simulink model "W06_1_point"  (R2024b)
settings: Solver=ode4  StartTime=0  StopTime=120  FixedStep=h  RelTol=1e-3
InitFcn:
  | addpath(fullfile(fileparts(fileparts(fileparts(get_param(bdroot, 'FileName')))), '_tools'), fileparts(get_param(bdroot, 'FileName'))); run_alone('W06', bdroot);
StopFcn:
  | W06_plot;
values from neighbouring files (symbols this model uses):
  animate = 1    [W06_0_setup.m]    (also in W06_1_point_run.m = 0; W06_2_sway_run.m = 0; W06_3_thrust_run.m = 0; W06_4_stop_run.m = 0)
  beta_c = pi/2    (= 1.57079632679)    [W06_0_setup.m]    (also in W06_4_stop_run.m = V.beta_c)
  Binv = inv(B)    [W06_0_setup.m]
  bow = [l_f, k_bow, n_bow_max]    [W06_0_setup.m]
  h = 0.02    [W06_0_setup.m]
  k_bow = cfg.k_bow    [W06_0_setup.m]
  k_neg = cfg.k_neg    [W06_0_setup.m]
  k_pos = cfg.k_pos    [W06_0_setup.m]
  Kb = 1    [W06_0_setup.m]
  Kd = 100    [W06_0_setup.m]
  Ki_u = 200    [W06_0_setup.m]
  Ki_v = 120    [W06_0_setup.m]
  Kp = 300    [W06_0_setup.m]
  Kp_pos = 0.30    (= 0.3)    [W06_0_setup.m]    (also in W06_4_stop_run.m = V.Kp_pos)
  Kp_u = 200    [W06_0_setup.m]
  Kp_v = 150    [W06_0_setup.m]
  mp = 25    [W06_0_setup.m]
  n_bow_max = cfg.n_bow_max    [W06_0_setup.m]    (also in W06_1_point_run.m = V.n_bow_max)
  n_max = cfg.n_max    [W06_0_setup.m]
  N_max = 2*y_pont*min(T_max, -T_min)    [W06_0_setup.m]
  n_min = cfg.n_min    [W06_0_setup.m]
  psi_d_cmd = 0    [W06_0_setup.m]    (also in W06_1_point_run.m; W06_8_ned_run.m)
  rp = [0.05 0 -0.35]'    [W06_0_setup.m]
  u_lim = 0.80    (= 0.8)    [W06_0_setup.m]
  V_c = 0    [W06_0_setup.m]    (also in W06_4_stop_run.m = V.V_c)
  v_lim = 0.35    [W06_0_setup.m]
  x0 = zeros(12,1)    [W06_0_setup.m]
  X_max = 120    [W06_0_setup.m]    (also in W06_plot.m = base_var('X_max', 120))
  Y_max = min(abs(T_min)/(l_f/(2*y_pont)), F_B_max)    [W06_0_setup.m]    (also in W06_plot.m = base_var('Y_max', 35.13))
settings Model: Creator=admin  LastModifiedBy=admin
settings DataIOCC: ReturnWorkspaceOutputs=off

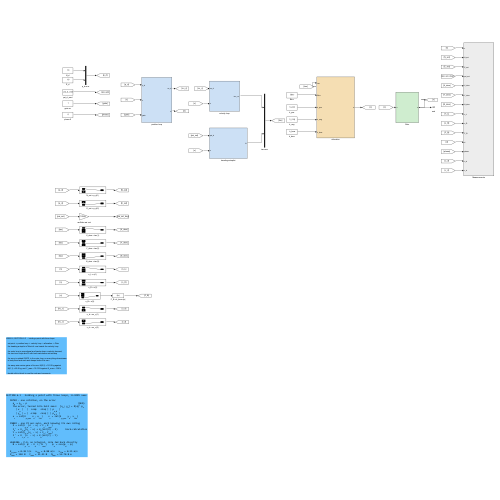
[thumbnail: Simulink's stored preview of the top-level diagram]
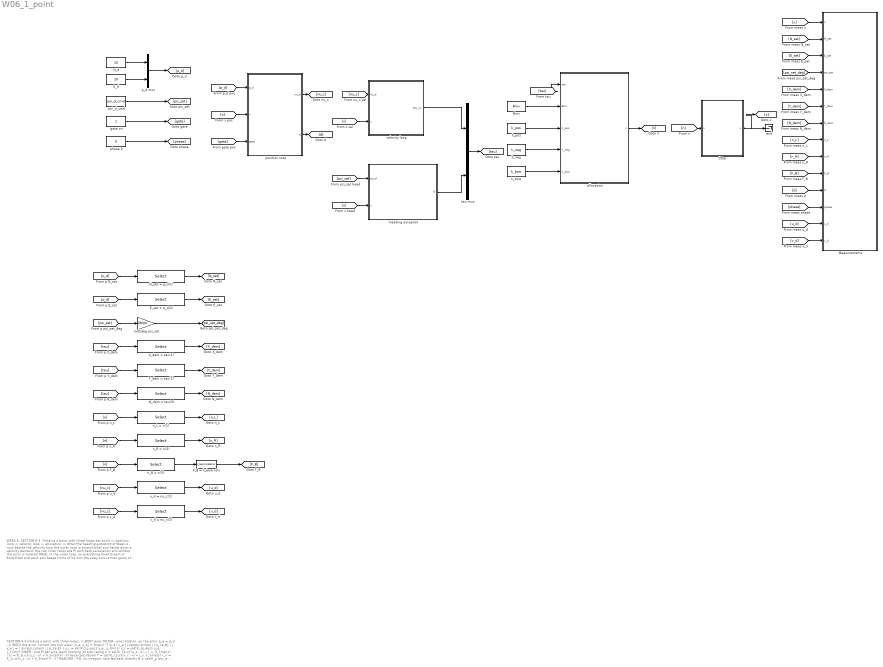
== system W06_1_point ==
  note: WEEK 6, SECTION 6-3  -  holding a point with three loops
      |
      |    set point -> position loop -> velocity loop -> allocation -> Otter
      |    the heading autopilot of Week 4 runs beside the velocity loop
      |
      |    the outer loop is proportional and hands down a velocity demand;
      |    the two inner loops are PI with back-calculation anti-windup
      |
      |    the error is rotated ONCE, in the outer loop, so everything downstream
      |    is body-fixed and each axis keeps limits of its own
      |
      |    the sway axis carries gains of its own: M(2,2) = 162.5 kg against
      |    M(1,1) = 85.5 kg, and Y_max = 35.13 N against X_max = 120 N
      |
      |    double-click a block to read its code and comments
  note: SECTION 6-3   holding a point with three loops, in BODY axes
      |
      |    OUTER - one rotation, on the error
      |      p_e = p_d - p                                      (NED)
      |      the error, turned into hull axes:  [x_e; y_e] = R(\psi)^T p_e
      |        | x_e |   |  cos\psi   sin\psi | | p_{e,N} |
      |        | y_e | = | -sin\psi   cos\psi | | p_{e,E} |
      |      u_c = sat(K_{p,pos} x_e, u_{lim})    v_c = sat(K_{p,pos} y_e, v_{lim})
      |
      |    INNER - one PI per axis, each knowing its own rating
      |      X = sat(K_{p,u}(u_c - u) + I_u, X_{max})
      |      I_u' = K_{i,u}(u_c - u) + K_b(sat(X) - X)      back-calculation
      |      Y = sat(K_{p,v}(v_c - v) + I_v, Y_{max})
      |      I_v' = K_{i,v}(v_c - v) + K_b(sat(Y) - Y)
      |
      |    HEADING - P-D, no integral, rate fed back directly
      |      N = sat(K_p \psi_e - K_d r, N_{max})    \psi_e = ssa(\psi_d - \psi)
      |
      |    K_{p,pos} = 0.30 1/s   u_{lim} = 0.80 m/s   v_{lim} = 0.35 m/s
      |    X_{max} = 120 N   Y_{max} = 35.13 N   N_{max} = 52.70 N m
  Binv : Constant  Value=Binv
  E_d : Constant  Value=10
  E_set = p_d(2) : Selector  InputPortWidth=2  IndexOptions=Index vector (dialog)  Indices=2  OutputSizes=1
  F_B = k_bow n|n| : Fcn  Expr=k_bow*u*abs(u)
  Measurements : Subsystem
  N_d : Constant  Value=10
  N_dem = tau(3) : Selector  InputPortWidth=3  IndexOptions=Index vector (dialog)  Indices=3  OutputSizes=1
  N_set = p_d(1) : Selector  InputPortWidth=2  IndexOptions=Index vector (dialog)  Indices=1  OutputSizes=1
  Otter : Subsystem
  X_dem = tau(1) : Selector  InputPortWidth=3  IndexOptions=Index vector (dialog)  Indices=1  OutputSizes=1
  Y_dem = tau(2) : Selector  InputPortWidth=3  IndexOptions=Index vector (dialog)  Indices=2  OutputSizes=1
  allocation : Subsystem
  end : Terminator
  gate on : Constant
  heading autopilot : Subsystem
  k_bow : Constant  Value=k_bow
  k_neg : Constant  Value=k_neg
  k_pos : Constant  Value=k_pos
  n_B = n(3) : Selector  InputPortWidth=3  IndexOptions=Index vector (dialog)  Indices=3  OutputSizes=1
  n_L = n(1) : Selector  InputPortWidth=3  IndexOptions=Index vector (dialog)  Indices=1  OutputSizes=1
  n_R = n(2) : Selector  InputPortWidth=3  IndexOptions=Index vector (dialog)  Indices=2  OutputSizes=1
  p_d mux : Mux  Inputs=2
  phase 0 : Constant  Value=0
  position loop : Subsystem
  psi_d_cmd : Constant  Value=psi_d_cmd
  rad2deg psi_set : Gain  Gain=180/pi
  tau mux : Mux  Inputs=2
  u_d = nu_c(1) : Selector  InputPortWidth=2  IndexOptions=Index vector (dialog)  Indices=1  OutputSizes=1
  v_d = nu_c(2) : Selector  InputPortWidth=2  IndexOptions=Index vector (dialog)  Indices=2  OutputSizes=1
  velocity loop : Subsystem
  wires:
  N_d/1 -> p_d mux/1
  E_d/1 -> p_d mux/2
  p_d mux/1 -> [p_d]
  psi_d_cmd/1 -> [psi_set]
  gate on/1 -> [gate]
  phase 0/1 -> [phase]
  [p_d] -> position loop/1(p_d)
  [x] -> position loop/2(x)
  [gate] -> position loop/3(gate)
  position loop/2(d) -> [d]
  position loop/1(nu_d) -> [nu_c]
  [nu_c] -> velocity loop/1(nu_d)
  [x] -> velocity loop/2(x)
  [psi_set] -> heading autopilot/1(psi_d)
  [x] -> heading autopilot/2(x)
  velocity loop/1(tau_uv) -> tau mux/1
  heading autopilot/1(N) -> tau mux/2
  tau mux/1 -> [tau]
  [tau] -> allocation/1(tau)
  Binv/1 -> allocation/2(Binv)
  k_pos/1 -> allocation/3(k_pos)
  k_neg/1 -> allocation/4(k_neg)
  k_bow/1 -> allocation/5(k_bow)
  allocation/1(n) -> [n]
  [n] -> Otter/1(n)
  Otter/1(x) -> [x], end/1
  [x] -> Measurements/1(x)
  [N_set] -> Measurements/2(N_set)
  [E_set] -> Measurements/3(E_set)
  [psi_set_deg] -> Measurements/4(psi_set)
  [X_dem] -> Measurements/5(X_dem)
  [Y_dem] -> Measurements/6(Y_dem)
  [N_dem] -> Measurements/7(N_dem)
  [n_L] -> Measurements/8(n_L)
  [n_R] -> Measurements/9(n_R)
  [F_B] -> Measurements/10(F_B)
  [d] -> Measurements/11(d)
  [phase] -> Measurements/12(phase)
  [u_d] -> Measurements/13(u_d)
  [v_d] -> Measurements/14(v_d)
  [p_d] -> N_set = p_d(1)/1
  N_set = p_d(1)/1 -> [N_set]
  [p_d] -> E_set = p_d(2)/1
  E_set = p_d(2)/1 -> [E_set]
  [psi_set] -> rad2deg psi_set/1
  rad2deg psi_set/1 -> [psi_set_deg]
  [tau] -> X_dem = tau(1)/1
  X_dem = tau(1)/1 -> [X_dem]
  [tau] -> Y_dem = tau(2)/1
  Y_dem = tau(2)/1 -> [Y_dem]
  [tau] -> N_dem = tau(3)/1
  N_dem = tau(3)/1 -> [N_dem]
  [n] -> n_L = n(1)/1
  n_L = n(1)/1 -> [n_L]
  [n] -> n_R = n(2)/1
  n_R = n(2)/1 -> [n_R]
  [n] -> n_B = n(3)/1
  n_B = n(3)/1 -> F_B = k_bow n|n|/1
  F_B = k_bow n|n|/1 -> [F_B]
  [nu_c] -> u_d = nu_c(1)/1
  u_d = nu_c(1)/1 -> [u_d]
  [nu_c] -> v_d = nu_c(2)/1
  v_d = nu_c(2)/1 -> [v_d]

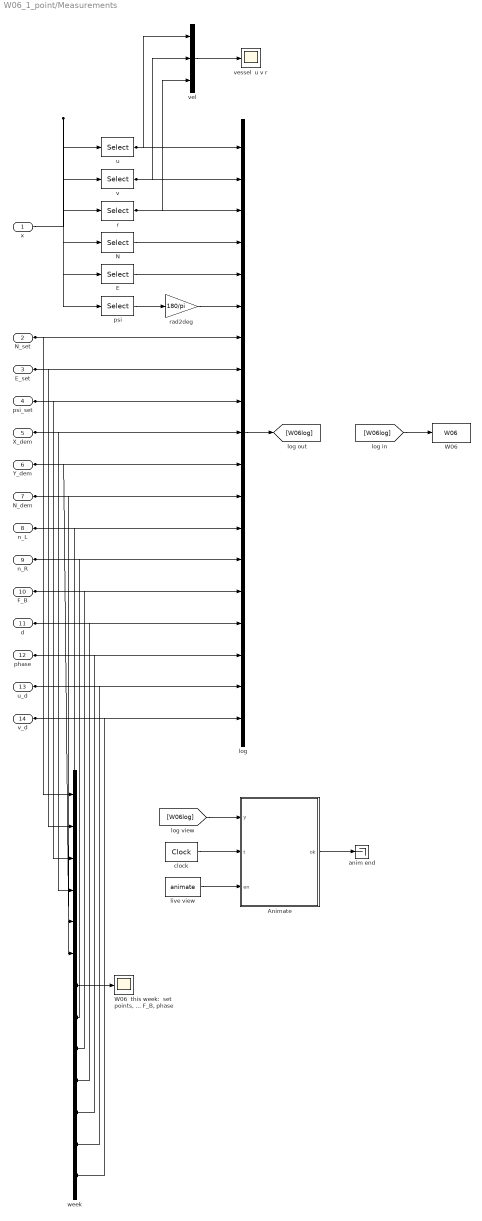
== system W06_1_point/Measurements ==
  x : Inport
  N_set : Inport  Port=2
  E_set : Inport  Port=3
  psi_set : Inport  Port=4
  X_dem : Inport  Port=5
  Y_dem : Inport  Port=6
  N_dem : Inport  Port=7
  n_L : Inport  Port=8
  n_R : Inport  Port=9
  F_B : Inport  Port=10
  d : Inport  Port=11
  phase : Inport  Port=12
  u_d : Inport  Port=13
  v_d : Inport  Port=14
  Animate : MATLAB Function  TreatAsAtomicUnit=on
  E : Selector  InputPortWidth=12  IndexOptions=Index vector (dialog)  Indices=8  OutputSizes=1
  N : Selector  InputPortWidth=12  IndexOptions=Index vector (dialog)  Indices=7  OutputSizes=1
  W06 : ToWorkspace  VariableName=W06  SaveFormat=Structure With Time  SampleTime=-1
  "W06  this week:  set points, demands, n_L n_R, F_B, phase" : Scope
  anim end : Terminator
  clock : DigitalClock  SampleTime=h
  live view : Constant  Value=animate
  log : Mux  Inputs=19
  psi : Selector  InputPortWidth=12  IndexOptions=Index vector (dialog)  Indices=12  OutputSizes=1
  r : Selector  InputPortWidth=12  IndexOptions=Index vector (dialog)  Indices=6  OutputSizes=1
  rad2deg : Gain  Gain=180/pi
  u : Selector  InputPortWidth=12  IndexOptions=Index vector (dialog)  Indices=1  OutputSizes=1
  v : Selector  InputPortWidth=12  IndexOptions=Index vector (dialog)  Indices=2  OutputSizes=1
  vel : Mux  Inputs=3
  vessel  u v r : Scope
  week : Mux  Inputs=13
  wires:
  x/1 -> u/1, v/1, r/1, N/1, E/1, psi/1
  log/1 -> [W06log]
  [W06log] -> W06/1
  psi/1 -> rad2deg/1
  u/1 -> log/1, vel/1
  v/1 -> log/2, vel/2
  r/1 -> log/3, vel/3
  N/1 -> log/4
  E/1 -> log/5
  rad2deg/1 -> log/6
  N_set/1 -> log/7, week/1
  E_set/1 -> log/8, week/2
  psi_set/1 -> log/9, week/3
  X_dem/1 -> log/10, week/4
  Y_dem/1 -> log/11, week/5
  N_dem/1 -> log/12, week/6
  n_L/1 -> log/13, week/7
  n_R/1 -> log/14, week/8
  F_B/1 -> log/15, week/9
  d/1 -> log/16, week/10
  phase/1 -> log/17, week/11
  u_d/1 -> log/18, week/12
  v_d/1 -> log/19, week/13
  vel/1 -> vessel  u v r/1
  week/1 -> "W06  this week:  set points, demands, n_L n_R, F_B, phase"/1
  [W06log] -> Animate/1(y)
  clock/1 -> Animate/2(t)
  live view/1 -> Animate/3(en)
  Animate/1(ok) -> anim end/1

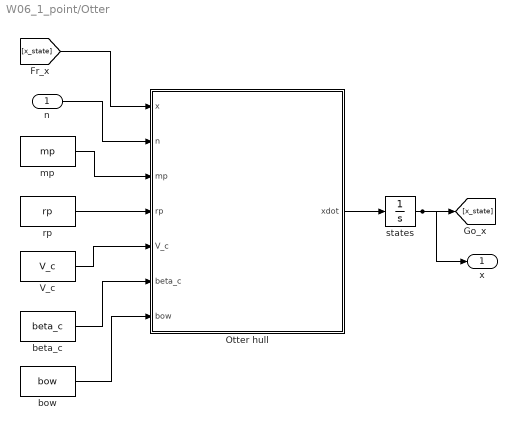
== system W06_1_point/Otter ==
  n : Inport
  Otter hull : MATLAB Function  TreatAsAtomicUnit=on
  V_c : Constant  Value=V_c
  beta_c : Constant  Value=beta_c
  bow : Constant  Value=bow
  mp : Constant  Value=mp
  rp : Constant  Value=rp
  states : Integrator  InitialCondition=x0
  x : Outport
  wires:
  [x_state] -> Otter hull/1(x)
  bow/1 -> Otter hull/7(bow)
  rp/1 -> Otter hull/4(rp)
  n/1 -> Otter hull/2(n)
  Otter hull/1(xdot) -> states/1
  mp/1 -> Otter hull/3(mp)
  V_c/1 -> Otter hull/5(V_c)
  beta_c/1 -> Otter hull/6(beta_c)
  states/1 -> [x_state], x/1

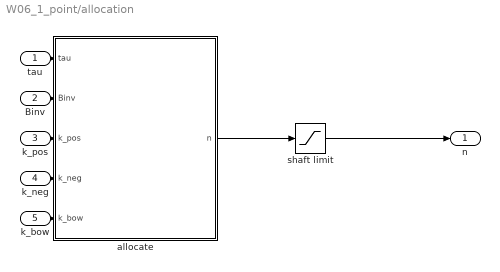
== system W06_1_point/allocation ==
  tau : Inport
  Binv : Inport  Port=2
  k_pos : Inport  Port=3
  k_neg : Inport  Port=4
  k_bow : Inport  Port=5
  allocate : MATLAB Function  TreatAsAtomicUnit=on
  shaft limit : Saturate  UpperLimit="[ n_max;  n_max;  n_bow_max]"  LowerLimit="[ n_min;  n_min; -n_bow_max]"
  n : Outport
  wires:
  tau/1 -> allocate/1(tau)
  Binv/1 -> allocate/2(Binv)
  k_pos/1 -> allocate/3(k_pos)
  k_neg/1 -> allocate/4(k_neg)
  k_bow/1 -> allocate/5(k_bow)
  allocate/1(n) -> shaft limit/1
  shaft limit/1 -> n/1

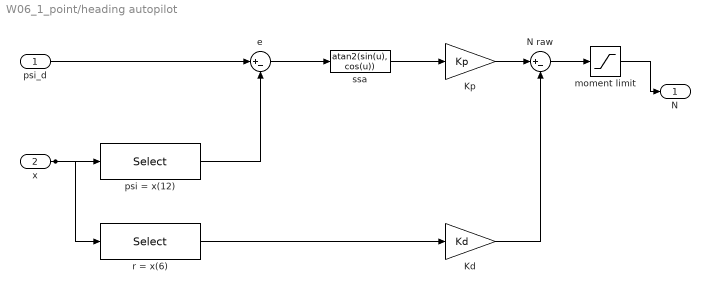
== system W06_1_point/heading autopilot ==
  psi_d : Inport
  x : Inport  Port=2
  Kd : Gain  Gain=Kd
  Kp : Gain  Gain=Kp
  N raw : Sum  Inputs=|+-
  e : Sum  Inputs=|+-
  moment limit : Saturate  UpperLimit=N_max  LowerLimit=-N_max
  psi = x(12) : Selector  InputPortWidth=12  IndexOptions=Index vector (dialog)  Indices=12  OutputSizes=1
  r = x(6) : Selector  InputPortWidth=12  IndexOptions=Index vector (dialog)  Indices=6  OutputSizes=1
  ssa : Fcn  Expr=atan2(sin(u), cos(u))
  N : Outport
  wires:
  x/1 -> psi = x(12)/1, r = x(6)/1
  psi_d/1 -> e/1
  psi = x(12)/1 -> e/2
  e/1 -> ssa/1
  ssa/1 -> Kp/1
  r = x(6)/1 -> Kd/1
  Kp/1 -> N raw/1
  Kd/1 -> N raw/2
  N raw/1 -> moment limit/1
  moment limit/1 -> N/1

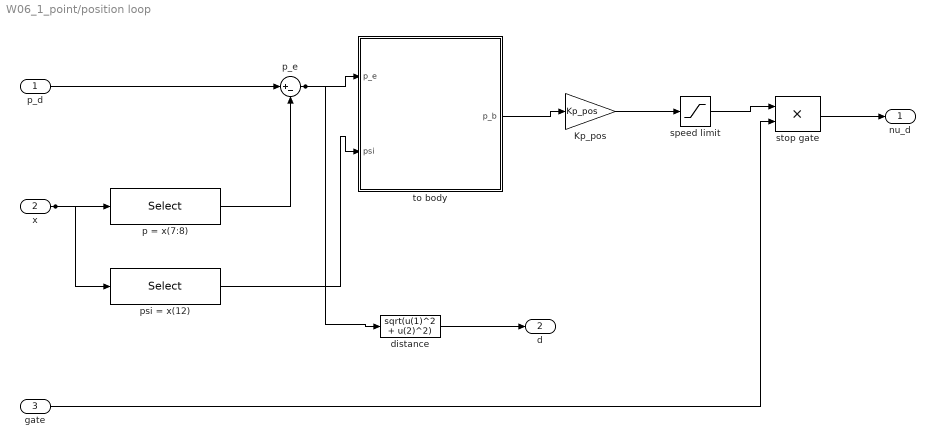
== system W06_1_point/position loop ==
  p_d : Inport
  x : Inport  Port=2
  gate : Inport  Port=3
  Kp_pos : Gain  Gain=Kp_pos
  distance : Fcn  Expr=sqrt(u(1)^2 + u(2)^2)
  p = x(7:8) : Selector  InputPortWidth=12  IndexOptions=Index vector (dialog)  Indices=[7 8]  OutputSizes=1
  p_e : Sum  Inputs=|+-
  psi = x(12) : Selector  InputPortWidth=12  IndexOptions=Index vector (dialog)  Indices=12  OutputSizes=1
  speed limit : Saturate  UpperLimit="[ u_lim;  v_lim]"  LowerLimit=[-u_lim; -v_lim]
  stop gate : Product
  to body : MATLAB Function  TreatAsAtomicUnit=on
  nu_d : Outport
  d : Outport  Port=2
  wires:
  x/1 -> p = x(7:8)/1, psi = x(12)/1
  p_d/1 -> p_e/1
  p = x(7:8)/1 -> p_e/2
  p_e/1 -> to body/1(p_e), distance/1
  psi = x(12)/1 -> to body/2(psi)
  to body/1(p_b) -> Kp_pos/1
  Kp_pos/1 -> speed limit/1
  speed limit/1 -> stop gate/1
  gate/1 -> stop gate/2
  stop gate/1 -> nu_d/1
  distance/1 -> d/1

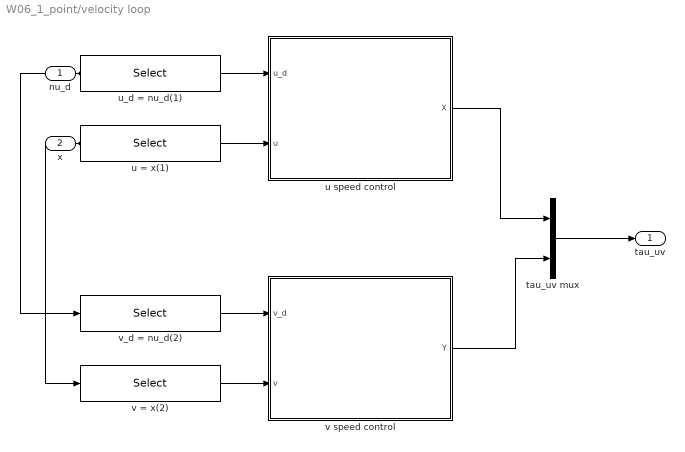
== system W06_1_point/velocity loop ==
  nu_d : Inport
  x : Inport  Port=2
  tau_uv mux : Mux  Inputs=2
  u = x(1) : Selector  InputPortWidth=12  IndexOptions=Index vector (dialog)  Indices=1  OutputSizes=1
  u speed control : Subsystem
  u_d = nu_d(1) : Selector  InputPortWidth=2  IndexOptions=Index vector (dialog)  Indices=1  OutputSizes=1
  v = x(2) : Selector  InputPortWidth=12  IndexOptions=Index vector (dialog)  Indices=2  OutputSizes=1
  v speed control : Subsystem
  v_d = nu_d(2) : Selector  InputPortWidth=2  IndexOptions=Index vector (dialog)  Indices=2  OutputSizes=1
  tau_uv : Outport
  wires:
  u_d = nu_d(1)/1 -> u speed control/1(u_d)
  u = x(1)/1 -> u speed control/2(u)
  v_d = nu_d(2)/1 -> v speed control/1(v_d)
  v = x(2)/1 -> v speed control/2(v)
  nu_d/1 -> u_d = nu_d(1)/1, v_d = nu_d(2)/1
  x/1 -> u = x(1)/1, v = x(2)/1
  u speed control/1(X) -> tau_uv mux/1
  v speed control/1(Y) -> tau_uv mux/2
  tau_uv mux/1 -> tau_uv/1

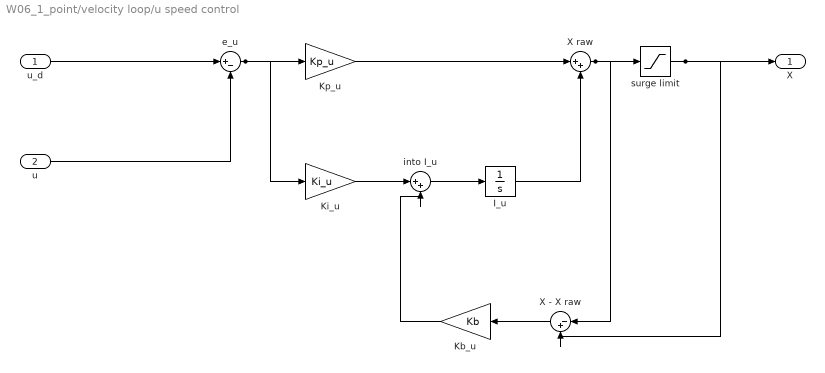
== system W06_1_point/velocity loop/u speed control ==
  u_d : Inport
  u : Inport  Port=2
  I_u : Integrator
  Kb_u : Gain  Gain=Kb
  Ki_u : Gain  Gain=Ki_u
  Kp_u : Gain  Gain=Kp_u
  X - X raw : Sum  Inputs=|-+
  X raw : Sum  Inputs=|++
  e_u : Sum  Inputs=|+-
  into I_u : Sum  Inputs=|++
  surge limit : Saturate  UpperLimit=X_max  LowerLimit=-X_max
  X : Outport
  wires:
  u_d/1 -> e_u/1
  u/1 -> e_u/2
  e_u/1 -> Kp_u/1, Ki_u/1
  Ki_u/1 -> into I_u/1
  into I_u/1 -> I_u/1
  Kp_u/1 -> X raw/1
  I_u/1 -> X raw/2
  X raw/1 -> surge limit/1, X - X raw/1
  surge limit/1 -> X - X raw/2, X/1
  X - X raw/1 -> Kb_u/1
  Kb_u/1 -> into I_u/2

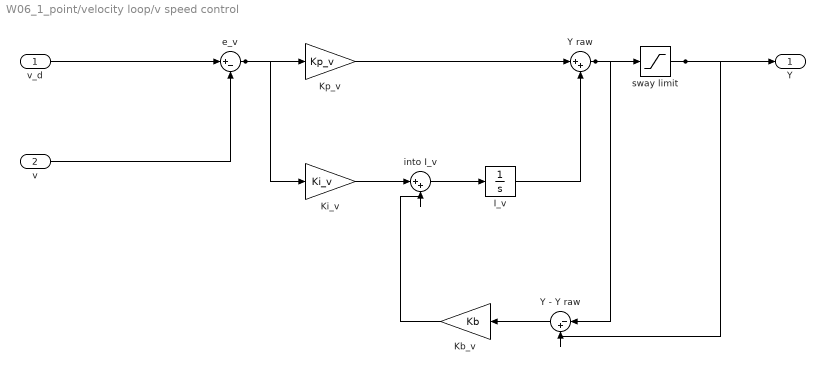
== system W06_1_point/velocity loop/v speed control ==
  v_d : Inport
  v : Inport  Port=2
  I_v : Integrator
  Kb_v : Gain  Gain=Kb
  Ki_v : Gain  Gain=Ki_v
  Kp_v : Gain  Gain=Kp_v
  Y - Y raw : Sum  Inputs=|-+
  Y raw : Sum  Inputs=|++
  e_v : Sum  Inputs=|+-
  into I_v : Sum  Inputs=|++
  sway limit : Saturate  UpperLimit=Y_max  LowerLimit=-Y_max
  Y : Outport
  wires:
  v_d/1 -> e_v/1
  v/1 -> e_v/2
  e_v/1 -> Kp_v/1, Ki_v/1
  Ki_v/1 -> into I_v/1
  into I_v/1 -> I_v/1
  Kp_v/1 -> Y raw/1
  I_v/1 -> Y raw/2
  Y raw/1 -> sway limit/1, Y - Y raw/1
  sway limit/1 -> Y - Y raw/2, Y/1
  Y - Y raw/1 -> Kb_v/1
  Kb_v/1 -> into I_v/2

== matlab function W06_1_point/allocation/allocate ==
  data: tau input; n output double size=[3 1]; Binv input; k_pos input; k_neg input; k_bow input
function n = allocate(tau, Binv, k_pos, k_neg, k_bow)
% Run the actuator model backwards: tau -> f -> u -> n.
%
%   forward    u_i = n_i|n_i|      f = K u        tau = B f
%   inverse    f = B^-1 tau        u = K^-1 f     n_i = sign(u_i) sqrt(|u_i|)
%
%   B    = [    1         1       0  ]    f   = [T_L; T_R; F_B]  [N]
%          [    0         0       1  ]    tau = [X; Y; N]        [N, N, N m]
%          [ y_pont   -y_pont   l_f ]
%
% B is square and non-singular (det B = 0.79), so the solution is unique and
% there is no null space to choose within. Binv comes from the setup script,
% which inverts the B that otter_B() derives from the column rule.
f = Binv * tau;

% K is diagonal, so K^-1 is three divisions. Which coefficient applies depends
% on the sign for a stern propeller, because a propeller pushing astern is
% less efficient than the same propeller pushing ahead. It does not depend on
% the sign for the bow unit: a tunnel thruster is symmetric.
k = [k_pos; k_pos; k_bow];
if f(1) < 0, k(1) = k_neg; end
if f(2) < 0, k(2) = k_neg; end

u = f ./ k;

% n_i = sign(u_i) sqrt(|u_i|). The absolute value is not decoration: slide 133
% writes sqrt(u_i), and without the |.| every astern command returns a complex
% shaft speed.
n = sign(u) .* sqrt(abs(u));
end

== matlab function W06_1_point/position loop/to body ==
  data: p_e input; p_b output double size=[2 1]; psi input
function p_b = to_body(p_e, psi)
% Rotate the position error from NED into the body frame.
%
%            [ cos(psi)  -sin(psi) ]
%   R(psi) = [ sin(psi)   cos(psi) ]     maps the BODY frame to NED,
%
% so the transpose maps NED to the body frame. R is orthogonal, so the
% transpose is the inverse and nothing is lost in the change of frame: the
% distance to the target is the same number in either one.
c = cos(psi);
s = sin(psi);
p_b = [  c*p_e(1) + s*p_e(2) ;      % 전진 방향의 오차 / along the bow
        -s*p_e(1) + c*p_e(2) ];     % 우현 방향의 오차 / to starboard
end

== matlab function W06_1_point/Otter/Otter hull ==
  data: x input; xdot output double size=[12 1]; n input; mp input; rp input; V_c input; beta_c input; bow input
function xdot = otter_hull(x, n, mp, rp, V_c, beta_c, bow)
% otter_bow.m: Fossen's otter.m with a bow tunnel thruster added, called
% unchanged from _tools. Three shaft speeds in, tau built inside.
%
%   x     12 states, fed back from the integrator
%   n     shaft speeds [rad/s]: port stern, starboard stern, bow
%   bow   [l3 k3 n3_max], the bow unit's arm, coefficient and speed limit
%
% The sway force and its moment are now rows 2 and 6 of the tau that the
% motion model builds for itself. Nothing is added after the call.
%
% otter_bow.m is not written for code generation, so the call is extrinsic
% and xdot has to be pre-sized for Simulink to know the output width.
coder.extrinsic('otter_bow');

xdot = zeros(12,1);
xdot = otter_bow(x, n, mp, rp, V_c, beta_c, bow);
end

== matlab function W06_1_point/Measurements/Animate ==
  data: y input; ok output; t input; en input
function ok = Animate(y, t, en)
%#codegen
% Live view of the vessel while the model runs.
%
% A MATLAB Function block cannot plot, so the drawing function is declared
% extrinsic: Simulink calls plain MATLAB rather than generating code for it.
% Set animate = 0 in the setup script to switch the live view off.
%
% y is the whole log vector, in the column order this subsystem builds:
% [u v r N E psi] first, psi in DEGREES, then the week's own signals.
% The wrapper names the columns; nothing else counts them.
coder.extrinsic('W06_animate');
ok = 1;
if en > 0.5
    W06_animate(y, t);
end
end
